simulink model "TAMRIN2"  (R2023b)
settings: Solver=VariableStepAuto  StartTime=0.0  StopTime=10.0  RelTol=1e-3
settings Model: Creator=hp  LastModifiedBy=hp

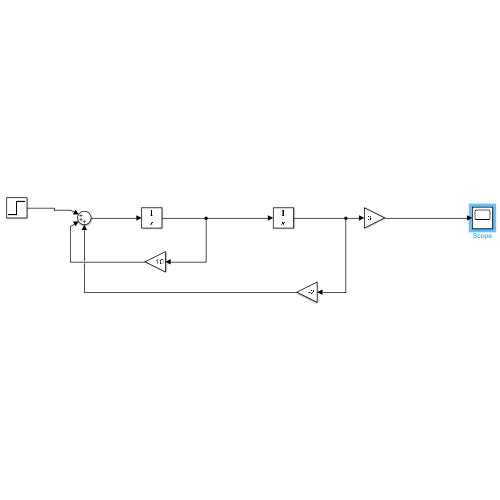
[thumbnail: Simulink's stored preview of the top-level diagram]
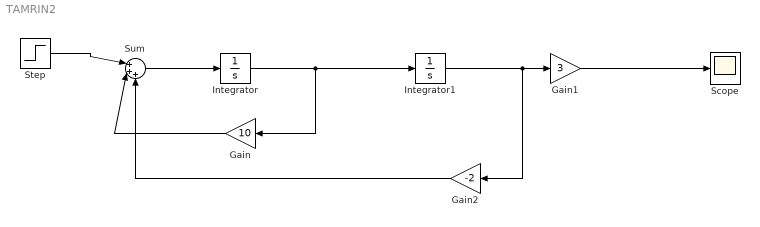
== system TAMRIN2 ==
  Gain : Gain  Gain=10
  Gain1 : Gain  Gain=3
  Gain2 : Gain  Gain=-2
  Integrator : Integrator  InitialCondition=20
  Integrator1 : Integrator
  Scope : Scope
  Step : Step  SampleTime=0
  Sum : Sum  Inputs=|+++
  wires:
  Integrator/1 -> Gain/1, Integrator1/1
  Step/1 -> Sum/1
  Sum/1 -> Integrator/1
  Gain/1 -> Sum/2
  Integrator1/1 -> Gain2/1, Gain1/1
  Gain1/1 -> Scope/1
  Gain2/1 -> Sum/3
